simulink model "FCSMPC_double_vector_2025b"  (R2025b)
settings: Solver=FixedStepDiscrete  StartTime=0.0  StopTime=2  FixedStep=SimulinkTs  RelTol=1e-3
PreLoadFcn:
  | % Verzeichnis des Modells zum MATLAB-Pfad hinzufügen
  | modelDir = fileparts(get_param(bdroot, 'FileName'));
  | addpath(modelDir);
  | 
  | % Nur der Dateiname – kein Pfad!
  | set_param(bdroot, 'DataDictionary', 'FOC_params.sldd');
model workspace (MAT data in the model file):
  Np : Simulink.Parameter (value not decoded)
values from neighbouring files (symbols this model uses):
  Filter_Current_FilterTimeConst = 3.3333333333333335E-5    [FOC_params.sldd]
  Filter_Current_SensorTimeConst = 1.5915494309189535E-6    [FOC_params.sldd]
  FOC = evalin("base", "FOC")    [createFOC_SLDD.m]
  FOC_Control_Current_KIid = 10.0    [FOC_params.sldd]
  FOC_Control_Current_KIiq = 10.0    [FOC_params.sldd]
  FOC_Control_Current_KPid = 0.20418507462686566    [FOC_params.sldd]
  FOC_Control_Current_KPiq = 0.58674626865671642    [FOC_params.sldd]
  FOC_Control_Current_Krd = 0.8    [FOC_params.sldd]
  FOC_Control_Current_Krq = 0.8    [FOC_params.sldd]
  FOC_Control_Current_TclCur = 0.1    [FOC_params.sldd]
  FOC_Control_Current_Tnd = 0.1    [FOC_params.sldd]
  FOC_Control_Current_Tnq = 0.1    [FOC_params.sldd]
  FOC_Control_InverterVdc_V = 400.0    [FOC_params.sldd]
  FOC_Control_MotorImax_A = 650.0    [FOC_params.sldd]
  FOC_Control_MTPA_MTPV_nT_id_grid = -450.06704889786266 -439.56177000270145 -427.77784873303676 -416.66404703197372 -406.07553272717422 -395.15516533678584 -384.31176061747851 -374.03652088128132 -363.90551910193739 -353.79478643334204 -344.0221683092833 -334.51243453441936 -324.94614350292119 -315.21793409137081 -305.26543360965195 -295.21828280911944 -285.133916324101 -275.01232812136521 -264.86951532374729 -254.7797625148454 -244    [FOC_params.sldd]
  FOC_Control_MTPA_MTPV_nT_iq_grid = -449.09165648258488 -442.56958748923387 -437.25247759546528 -430.91792082419158 -423.83735797306491 -417.11730433547 -410.54064621830616 -403.71584331167304 -396.93611069310379 -390.15794305727007 -382.97216593027133 -375.44639668848538 -367.93447385667577 -360.57088856352266 -353.41289778449368 -346.34020584402072 -339.28416684923008 -332.22010880540631 -325.11927997033376 -317.92299905654966 -31    [FOC_params.sldd]
  FOC_Control_MTPA_MTPV_T_vec = -245.0 -240.0 -235.0 -230.0 -225.0 -220.0 -215.0 -210.0 -205.0 -200.0 -195.0 -190.0 -185.0 -180.0 -175.0 -170.0 -165.0 -160.0 -155.0 -150.0 -145.0 -140.0 -135.0 -130.0 -125.0 -120.0 -115.0 -110.0 -105.0 -100.0 -95.0 -90.0 -85.0 -80.0 -75.0 -70.0 -65.0 -60.0 -55.0 -50.0 -45.0 -40.0 -35.0 -30.0 -25.0 -20.0 -15.0 -10.0 -5.0 0.0 5.0 10.0 15.0 20.0 25.0 30.0 35.0 40.0 45.0 50.0 55.0 60.0 65.0 70.0 75.0    [FOC_params.sldd]
  FOC_Control_MTPA_MTPV_w_vec = 0.0 10.471975511965978 20.943951023931955 31.415926535897931 41.887902047863911 52.359877559829883 62.831853071795862 73.303828583761828 83.775804095727821 94.247779607693786 104.71975511965977 115.19173063162575 125.66370614359172 136.1356816555577 146.60765716752366 157.07963267948966 167.55160819145564 178.02358370342159 188.49555921538757 198.96753472735358 209.43951023931953 219.9114857512855    [FOC_params.sldd]
  FOC_Control_OpenLoop_Id_Ref_A = 0.0    [FOC_params.sldd]
  FOC_Control_OpenLoop_Iq_Ref_A = 0.0    [FOC_params.sldd]
  FOC_Control_OpenLoop_Ud_OpenLoop_V = 0.0    [FOC_params.sldd]
  FOC_Control_OpenLoop_Uq_OpenLoop_V = 0.0    [FOC_params.sldd]
  FOC_Control_RF_omegamech_rad_s = 3141.5926535897934    [FOC_params.sldd]
  FOC_Control_RF_RateCurrent_A = 500.0    [FOC_params.sldd]
  FOC_Control_RF_RateTrq_Nm = 500.0    [FOC_params.sldd]
  FOC_Control_theta_mechOffsetFix = 0.0    [FOC_params.sldd]
  FOC_Control_theta_mechOffsetTime = 0.0    [FOC_params.sldd]
  FOC_Control_TorqueRef_Nm = 10.0    [FOC_params.sldd]
  FOC_Control_Umax_V = 230.94010767585033    [FOC_params.sldd]
  FOC_Flag_ClosedLoopControl = 1.0    [FOC_params.sldd]
  FOC_Flag_ControlStrategy = 2.0    [FOC_params.sldd]
  FOC_Flag_PWMEnable = 1.0    [FOC_params.sldd]
  FOC_Flag_ResetControl = 0.0    [FOC_params.sldd]
  FOC_Flag_TorqueControl = 1.0    [FOC_params.sldd]
  FOC_LUT_DQLimiter_DQ_LUTScaling = 1.8749999999999995E-5    [FOC_params.sldd]
  FOC_PWM_AZSPWMMethod = 3.0    [FOC_params.sldd]
  FOC_PWM_HybridMode = 1.0    [FOC_params.sldd]
  FOC_PWM_LB1 = 0.5    [FOC_params.sldd]
  FOC_PWM_LB2 = 0.77    [FOC_params.sldd]
  FOC_PWM_PWMManuel = 1.0    [FOC_params.sldd]
  FOC_PWM_RSPWMMethod = 2.0    [FOC_params.sldd]
  FOC_PWM_UB1 = 0.66    [FOC_params.sldd]
  FOC_PWM_UB2 = 0.9    [FOC_params.sldd]
  FOC_SampleTime_TsCur = 0.0001    [FOC_params.sldd]
undefined symbols (not defined in the file or in its folder): dspblkCoreblockFVToolHelper, FCS, Filter, gcbh, Plant, SimulinkTs
libraries: hdlsllib x2, simulink x2, autolibfluxpmsm x1
(part 6 of 8)

== matlab function FCSMPC_double_vector_2025b/FCS_MPC/SDA_Solve/SDA Solve/PSPL_TestFrame/SDA_PL_Framework/QuadraticCalc ==
  data: problem input Bus: SdaProblemBus size=[1 1]; done output boolean size=[1 1]; start input boolean size=[1 1]; level input uint8 size=[1 1]; memory input Bus: SdaMemoryBus size=[1 1]; valid output boolean size=[1 1]; metricNew output double size=[1 1]; head output double size=[1 1]; center output double size=[1 1]; firstCandidate output boolean size=[1 1]; candidate output boolean size=[1 1]; residual output double size=[1 1]
function [done, valid, metricNew, head, center, firstCandidate, candidate, residual] = QuadraticCalc(problem, start, level, memory)
%#codegen
persistent metricReg headReg centerReg firstReg candidateReg residualReg validReg
if isempty(metricReg)
    metricReg=0.0; headReg=0.0; centerReg=0.0;
    firstReg=false; candidateReg=false; residualReg=0.0; validReg=false;
end
done=false;
if start
    idx=max(uint8(1),min(uint8(15),level));
    row=double(idx); headReg=0.0;
    for k=1:15
        if k<row
            headReg=headReg+problem.H(row,k)*double(memory.Uwork(k));
        end
    end
    diagonal=problem.H(row,row);
    validReg=isfinite(diagonal)&&abs(diagonal)>1e-12;
    if validReg
        centerReg=(memory.z(row)-headReg)/diagonal;
        firstReg=centerReg>0.5;
        if memory.candidatePosition(row)==uint8(1)
            candidateReg=firstReg;
        else
            candidateReg=~firstReg;
        end
        residualReg=memory.z(row)-headReg-diagonal*double(candidateReg);
        metricReg=memory.metricStack(row)+residualReg*residualReg;
        validReg=isfinite(centerReg)&&isfinite(metricReg);
    else
        centerReg=0.0; firstReg=false; candidateReg=false;
        residualReg=0.0; metricReg=realmax;
    end
    done=true;
end
valid=validReg; metricNew=metricReg; head=headReg; center=centerReg;
firstCandidate=firstReg; candidate=candidateReg; residual=residualReg;
end

== matlab function FCSMPC_double_vector_2025b/FCS_MPC/SDA_Solve/SDA Solve/PSPL_TestFrame/SDA_PL_Framework/ResultCommit ==
  data: problem input Bus: SdaProblemBus size=[1 1]; result output Bus: SdaResultBus size=[1 1]; commit input boolean size=[1 1]; best input Bus: SdaBestBus size=[1 1]; nodes input uint32 size=[1 1]; leafNodes input uint32 size=[1 1]; nodeLimitReached input boolean size=[1 1]; Jround input double size=[1 1]; Jshift input double size=[1 1]
function result = ResultCommit(problem,commit,best,nodes,leafNodes,nodeLimitReached,Jround,Jshift)
%#codegen
persistent state
if isempty(state)
 state.valid=false; state.Jopt=realmax; state.nodes=uint32(0);
 state.optimal=false; state.Uopt=zeros(15,1); state.Uapply=zeros(6,1);
 state.leafNodes=uint32(0); state.bestCMVCost=0.0; state.cmvMetricRatio=0.0;
 state.switchCountApplied=uint32(0); state.debugLower=zeros(3,1);
 state.debugUpper=zeros(3,1); state.iabcPredictedNext=zeros(3,1);
 state.Jround=0.0; state.Jshift=0.0; state.predictionValidNext=false; state.solutionToggle=false;
end
if commit
 state.valid=best.bestValid; state.Jopt=best.bestMetric;
 state.nodes=nodes; state.leafNodes=leafNodes;
 state.optimal=best.bestValid&&~nodeLimitReached;
 state.Uopt=double(best.bestU); state.Uapply=state.Uopt(1:6);
 state.bestCMVCost=best.bestCMVCost;
 if state.Jopt>eps, state.cmvMetricRatio=state.bestCMVCost/state.Jopt; else, state.cmvMetricRatio=0.0; end
 sPrev=problem.UoptPrev(4:6); sFirst=state.Uopt(1:3); sSecond=state.Uopt(4:6);
 [deltaFirst,deltaDead]=deadtime_step(sPrev,sFirst,problem.iabcCompensated,problem);
 iabcAfter=problem.iabcCompensated+deltaFirst;
 [deltaSecond,~]=deadtime_step(sFirst,sSecond,iabcAfter,problem);
 state.iabcPredictedNext=iabcAfter+deltaSecond;
 state.switchCountApplied=uint32(sum(abs(sFirst-sPrev))+sum(abs(sSecond-sFirst)));
 [~,state.debugLower,state.debugUpper]=cmv_bounds(problem.iabcCompensated,deltaDead,problem.currentEpsMargin);
 state.Jround=Jround; state.Jshift=Jshift; state.predictionValidNext=best.bestValid;
 state.solutionToggle=~state.solutionToggle;
end
result=state;
end

function [deltaStep,deltaDead]=deadtime_step(sPrevious,sCurrent,iabc,problem)
sDead=sCurrent; signEps=0.1*problem.currentEpsMargin;
for phase=1:3
 if sPrevious(phase)~=sCurrent(phase)
  if iabc(phase)>=signEps, sDead(phase)=0.0;
  elseif iabc(phase)<=-signEps, sDead(phase)=1.0;
  elseif signEps>0.0, sDead(phase)=0.5*(1.0-iabc(phase)/signEps);
  else, sDead(phase)=0.5; end
 end
end
sEffective=problem.deadtimeRatio*sDead+(1.0-problem.deadtimeRatio)*sCurrent;
deltaDead=problem.deadtimeRatio*(problem.deltaIabcBase+problem.deltaIabcSwitch*sDead);
deltaStep=problem.deltaIabcBase+problem.deltaIabcSwitch*sEffective;
end

function [iabcEnd,lower,upper]=cmv_bounds(iabc,deltaDead,margin)
iabcEnd=iabc+deltaDead; lower=min(iabc,iabcEnd)-margin; upper=max(iabc,iabcEnd)+margin;
end

== matlab function FCSMPC_double_vector_2025b/FCS_MPC/SDA_Solve/SDA Solve/PSPL_TestFrame/SDA_PL_Framework/SdaInitializer ==
  data: problem input Bus: SdaProblemBus size=[1 1]; done output boolean size=[1 1]; start input boolean size=[1 1]; valid output boolean size=[1 1]; z output double size=[15 1]; initialU output double size=[15 1]; initialMetric output double size=[1 1]; initialCMVCost output double size=[1 1]; Jround output double size=[1 1]; Jshift output double size=[1 1]
function [done, valid, z, initialU, initialMetric, initialCMVCost, Jround, Jshift] = SdaInitializer(problem, start)
%#codegen
persistent zReg uReg metricReg cmvReg jRoundReg jShiftReg validReg
if isempty(zReg)
    zReg=zeros(15,1); uReg=zeros(15,1); metricReg=realmax;
    cmvReg=0.0; jRoundReg=0.0; jShiftReg=0.0; validReg=false;
end
done=false;
if start
    zReg=problem.H*problem.U_unc;
    uRound=zeros(15,1); uShift=zeros(15,1);
    for k=1:15
        uRound(k)=min(max(round(problem.U_unc(k)),0.0),1.0);
    end
    for k=1:12
        uShift(k)=problem.UoptPrev(k+3);
    end
    for k=13:15
        uShift(k)=problem.UoptPrev(k);
    end
    jRoundReg=quadratic_cost(problem.H,uRound,problem.U_unc);
    jShiftReg=quadratic_cost(problem.H,uShift,problem.U_unc);
    if jShiftReg < jRoundReg
        uReg=uShift;
    else
        uReg=uRound;
    end
    sPrevious=problem.UoptPrev(4:6);
    cmvReg=sequence_cmv_cost(uReg,sPrevious,problem);
    metricReg=quadratic_cost(problem.H,uReg,problem.U_unc)+cmvReg;
    validReg=isfinite(metricReg);
    done=true;
end
valid=validReg; z=zReg; initialU=uReg; initialMetric=metricReg;
initialCMVCost=cmvReg; Jround=jRoundReg; Jshift=jShiftReg;
end

function value=quadratic_cost(H,U,Uunc)
residual=H*(U-Uunc);
value=norm(residual,2)^2;
end

function total=sequence_cmv_cost(U,sPrevious,problem)
total=0.0; iabc=problem.iabcCompensated;
for step=1:5
    first=(step-1)*3+1; sCurrent=U(first:first+2);
    [deltaStep,deltaDead]=deadtime_step(sPrevious,sCurrent,iabc,problem);
    total=total+cmv_penalty(sPrevious,sCurrent,iabc,deltaDead,problem);
    iabc=iabc+deltaStep; sPrevious=sCurrent;
end
end

function [deltaStep,deltaDead]=deadtime_step(sPrevious,sCurrent,iabc,problem)
sDead=sCurrent; signEps=0.1*problem.currentEpsMargin;
for phase=1:3
    if sPrevious(phase)~=sCurrent(phase)
        if iabc(phase)>=signEps
            sDead(phase)=0.0;
        elseif iabc(phase)<=-signEps
            sDead(phase)=1.0;
        elseif signEps>0.0
            sDead(phase)=0.5*(1.0-iabc(phase)/signEps);
        else
            sDead(phase)=0.5;
        end
    end
end
sEffective=problem.deadtimeRatio*sDead+(1.0-problem.deadtimeRatio)*sCurrent;
deltaDead=problem.deadtimeRatio*(problem.deltaIabcBase+problem.deltaIabcSwitch*sDead);
deltaStep=problem.deltaIabcBase+problem.deltaIabcSwitch*sEffective;
end

function penalty=cmv_penalty(sPrevious,sCurrent,iabc,deltaDead,problem)
penalty=0.0; iabcEnd=iabc+deltaDead;
lower=min(iabc,iabcEnd)-problem.currentEpsMargin;
upper=max(iabc,iabcEnd)+problem.currentEpsMargin;
uncertain=(lower<=0.0)&(upper>=0.0);
if all(sCurrent==0.0)||all(sCurrent==1.0)
    penalty=penalty+problem.lambdaZero;
end
changed=(sPrevious~=sCurrent);
if sum(changed)~=2
    return;
end
canZero=false(3,1); canOne=false(3,1);
for phase=1:3
    if ~changed(phase)
        canZero(phase)=sPrevious(phase)==0.0;
        canOne(phase)=sPrevious(phase)==1.0;
    elseif uncertain(phase)
        canZero(phase)=true; canOne(phase)=true;
    elseif iabcEnd(phase)>0.0
        canZero(phase)=true;
    else
        canOne(phase)=true;
    end
end
if all(canZero)||all(canOne)
    penalty=penalty+problem.lambdaDeadtime;
end
end

== matlab function FCSMPC_double_vector_2025b/FCS_MPC/SDA_Solve/SDA Solve/PSPL_TestFrame/SDA_PL_Framework/SearchCounter ==
  data: clear input boolean size=[1 1]; nodes output uint32 size=[1 1]; writeEnable input boolean size=[1 1]; fsmState input uint8 size=[1 1]; level input uint8 size=[1 1]; problem input Bus: SdaProblemBus size=[1 1]; leafNodes output uint32 size=[1 1]; nodeLimitReached output boolean size=[1 1]; currentPrune input boolean size=[1 1]
function [nodes,leafNodes,nodeLimitReached] = SearchCounter(clear,writeEnable,fsmState,level,problem,currentPrune)
%#codegen
persistent nodeReg leafReg limitReg leafStatePrev
if isempty(nodeReg), nodeReg=uint32(0); leafReg=uint32(0); limitReg=false; leafStatePrev=false; end
if clear, nodeReg=uint32(0); leafReg=uint32(0); limitReg=false; leafStatePrev=false; end
if writeEnable&&fsmState==uint8(7)
 nodeReg=nodeReg+uint32(1);
 if problem.NmaxNode>uint32(0)&&nodeReg>problem.NmaxNode, limitReg=true; end
end
leafStateNow=fsmState==uint8(16);
if leafStateNow&&~leafStatePrev&&level==uint8(15)&&~currentPrune
 leafReg=leafReg+uint32(1);
end
leafStatePrev=leafStateNow;
nodes=nodeReg; leafNodes=leafReg; nodeLimitReached=limitReg;
end

== stateflow chart FCSMPC_double_vector_2025b/FCS_MPC/SDA_Solve/SDA Solve/PSPL_TestFrame/SDA_PL_Framework/SearchFSM ==
  settings: updateMethod=DISCRETE
  state IDLE
    entry: level=uint8(1); candidate=false; cycleCount=uint32(0); busy=false; resultValid=false; fault=false;
  state DONE
    entry: loadProblem=false; initStart=false; quadStart=false; vectorStart=false; memClear=false; memWrite=false; bestWrite=false; commitResult=false; busy=false; resultValid=true; fault=false;
  state FAULT
    entry: busy=false; fault=true;
  state LOAD
    entry: busy=true; loadProblem=true; memClear=true; level=uint8(1); cycleCount=uint32(0);
  state CENTER_WAIT
    during: loadProblem=false; initStart=false; quadStart=false; vectorStart=false; memClear=false; memWrite=false; bestWrite=false; commitResult=false; resultValid=false; fault=false; fsmState=uint8(6); cycleCount=cycleCount+uint32(1);
  state WRITE_RESULT
    entry: commitResult=true;
  state INIT_START
    entry: initStart=true;
  state INIT_WAIT
    during: loadProblem=false; initStart=false; quadStart=false; vectorStart=false; memClear=false; memWrite=false; bestWrite=false; commitResult=false; resultValid=false; fault=false; fsmState=uint8(3); cycleCount=cycleCount+uint32(1);
  state CENTER_START
    entry: quadStart=true;
  state SELECT_CANDIDATE
    entry: fsmState=uint8(7); candidate=quadCandidate; memWrite=true;
  state BACKTRACK
    entry: fsmState=uint8(17); if level>uint8(0); level=level-uint8(1); end; memWrite=true;
  state CHECK_LEVEL
    entry: loadProblem=false; initStart=false; quadStart=false; vectorStart=false; memClear=false; memWrite=false; bestWrite=false; commitResult=false; resultValid=false; fault=false; fsmState=uint8(4); cycleCount=cycleCount+uint32(1);
  state VECTOR_WAIT
    during: loadProblem=false; initStart=false; quadStart=false; vectorStart=false; memClear=false; memWrite=false; bestWrite=false; commitResult=false; resultValid=false; fault=false; fsmState=uint8(12); cycleCount=cycleCount+uint32(1);
  state NEXT_CANDIDATE
    entry: loadProblem=false; initStart=false; quadStart=false; vectorStart=false; memClear=false; memWrite=false; bestWrite=false; commitResult=false; resultValid=false; fault=false; fsmState=uint8(16); cycleCount=cycleCount+uint32(1);
  state DESCEND
    entry: fsmState=uint8(15); level=level+uint8(1); memWrite=true;
  state VECTOR_START
    entry: vectorStart=true;
  state VECTOR_CHECK
    entry: loadProblem=false; initStart=false; quadStart=false; vectorStart=false; memClear=false; memWrite=false; bestWrite=false; commitResult=false; resultValid=false; fault=false; fsmState=uint8(10); cycleCount=cycleCount+uint32(1);
  state UPDATE_BEST
    entry: bestWrite=true;
  state COMPARE
    entry: loadProblem=false; initStart=false; quadStart=false; vectorStart=false; memClear=false; memWrite=false; bestWrite=false; commitResult=false; resultValid=false; fault=false; fsmState=uint8(13); cycleCount=cycleCount+uint32(1);
  (default) -> IDLE
  DONE -> IDLE
  FAULT -> IDLE : [~start]
  IDLE -> LOAD : [start]
  CENTER_WAIT -> FAULT [order 2] : [quadDone && ~quadValid]
  WRITE_RESULT -> DONE
  INIT_WAIT -> FAULT [order 2] : [initDone && ~initValid]
  VECTOR_WAIT -> FAULT [order 2] : [vectorDone && ~vectorValid]
  LOAD -> INIT_START
  CENTER_WAIT -> SELECT_CANDIDATE [order 1] : [quadDone && quadValid]
  CENTER_START -> CENTER_WAIT
  INIT_START -> INIT_WAIT
  BACKTRACK -> WRITE_RESULT [order 2] : [level==uint8(0)]
  CHECK_LEVEL -> WRITE_RESULT [order 3] : [nodeLimitReached]
  INIT_WAIT -> CHECK_LEVEL [order 1] : [initDone && initValid]
  SELECT_CANDIDATE -> VECTOR_CHECK
  CHECK_LEVEL -> CENTER_START [order 1] : [~nodeLimitReached && ~candidateExhausted]
  CHECK_LEVEL -> BACKTRACK [order 2] : [~nodeLimitReached && candidateExhausted]
  BACKTRACK -> CHECK_LEVEL [order 1] : [level>uint8(0)]
  NEXT_CANDIDATE -> CHECK_LEVEL
  DESCEND -> CHECK_LEVEL
  VECTOR_WAIT -> COMPARE [order 1] : [vectorDone && vectorValid]
  VECTOR_START -> VECTOR_WAIT
  COMPARE -> NEXT_CANDIDATE [order 3] : [currentPrune || (level==uint8(15) && ~currentBetter)]
  UPDATE_BEST -> NEXT_CANDIDATE
  COMPARE -> DESCEND [order 2] : [level<uint8(15) && ~currentPrune]
  VECTOR_CHECK -> VECTOR_START [order 1] : [mod(level,uint8(3))==0]
  VECTOR_CHECK -> COMPARE [order 2] : [mod(level,uint8(3))~=0]
  COMPARE -> UPDATE_BEST [order 1] : [level==uint8(15) && currentBetter]
  data: start input boolean size=[1 1]; initDone input boolean size=[1 1]; initValid input boolean size=[1 1]; quadDone input boolean size=[1 1]; quadValid input boolean size=[1 1]; vectorDone input boolean size=[1 1]; vectorValid input boolean size=[1 1]; loadProblem output boolean size=[1 1]; initStart output boolean size=[1 1]; quadStart output boolean size=[1 1]; vectorStart output boolean size=[1 1]; memClear output boolean size=[1 1]; memWrite output boolean size=[1 1]; bestWrite output boolean size=[1 1]; commitResult output boolean size=[1 1]; busy output boolean size=[1 1]; resultValid output boolean size=[1 1]; fault output boolean size=[1 1]; level output uint8 size=[1 1]; candidate output boolean size=[1 1]; fsmState output uint8 size=[1 1]; cycleCount output uint32 size=[1 1]; quadCandidate input boolean size=[1 1]; candidateExhausted input boolean size=[1 1]; currentBetter input boolean size=[1 1]; currentPrune input boolean size=[1 1]; nodeLimitReached input boolean size=[1 1]

== matlab function FCSMPC_double_vector_2025b/FCS_MPC/SDA_Solve/SDA Solve/PSPL_TestFrame/SDA_PL_Framework/VectorCostCalc ==
  data: problem input Bus: SdaProblemBus size=[1 1]; done output boolean size=[1 1]; start input boolean size=[1 1]; level input uint8 size=[1 1]; memory input Bus: SdaMemoryBus size=[1 1]; valid output boolean size=[1 1]; totalMetricNew output double size=[1 1]; cmvMetricNew output double size=[1 1]; cmvIncrement output double size=[1 1]; iabcNext output double size=[3 1]; deltaStep output double size=[3 1]; deltaDead output double size=[3 1]; lowerBound output double size=[3 1]; upperBound output double size=[3 1]; deadtimeMiss output boolean size=[1 1]
function [done,valid,totalMetricNew,cmvMetricNew,cmvIncrement,iabcNext,deltaStep,deltaDead,lowerBound,upperBound,deadtimeMiss] = VectorCostCalc(problem,start,level,memory)
%#codegen
persistent totalReg cmvTotalReg incrementReg iabcReg stepReg deadReg lowerReg upperReg missReg validReg startPrev doneReg
if isempty(totalReg)
    totalReg=0.0; cmvTotalReg=0.0; incrementReg=0.0;
    iabcReg=zeros(3,1); stepReg=zeros(3,1); deadReg=zeros(3,1);
    lowerReg=zeros(3,1); upperReg=zeros(3,1);
    missReg=false; validReg=false; startPrev=false; doneReg=false;
end
done=doneReg;
if start&&~startPrev
    idx=max(uint8(3),min(uint8(15),level));
    predictionStep=idivide(idx,uint8(3));
    blockEnd=double(idx); blockStart=blockEnd-2;
    sCurrent=zeros(3,1); sPrevious=zeros(3,1);
    for phase=1:3
        sCurrent(phase)=double(memory.Uwork(blockStart+phase-1));
    end
    if predictionStep==uint8(1)
        sPrevious=problem.UoptPrev(4:6);
    else
        previousStart=blockStart-3;
        for phase=1:3
            sPrevious(phase)=double(memory.Uwork(previousStart+phase-1));
        end
    end
    iabcBefore=memory.iabcPrediction(:,double(predictionStep));
    [stepReg,deadReg]=deadtime_step(sPrevious,sCurrent,iabcBefore,problem);
    [incrementReg,lowerReg,upperReg,missReg]=cmv_penalty(sPrevious,sCurrent,iabcBefore,deadReg,problem);
    totalReg=memory.metricStack(double(idx)+1)+incrementReg;
    cmvTotalReg=memory.cmvMetricStack(double(idx))+incrementReg;
    iabcReg=iabcBefore+stepReg;
    validReg=all(isfinite(iabcReg))&&isfinite(totalReg)&&isfinite(cmvTotalReg);
    doneReg=true;
end
if ~start&&~startPrev, doneReg=false; end
startPrev=start;
valid=validReg; totalMetricNew=totalReg; cmvMetricNew=cmvTotalReg;
cmvIncrement=incrementReg; iabcNext=iabcReg; deltaStep=stepReg;
deltaDead=deadReg; lowerBound=lowerReg; upperBound=upperReg;
deadtimeMiss=missReg;
end

function [deltaStep,deltaDead]=deadtime_step(sPrevious,sCurrent,iabc,problem)
sDead=sCurrent; signEps=0.1*problem.currentEpsMargin;
for phase=1:3
    if sPrevious(phase)~=sCurrent(phase)
        if iabc(phase)>=signEps
            sDead(phase)=0.0;
        elseif iabc(phase)<=-signEps
            sDead(phase)=1.0;
        elseif signEps>0.0
            sDead(phase)=0.5*(1.0-iabc(phase)/signEps);
        else
            sDead(phase)=0.5;
        end
    end
end
sEffective=problem.deadtimeRatio*sDead+(1.0-problem.deadtimeRatio)*sCurrent;
deltaDead=problem.deadtimeRatio*(problem.deltaIabcBase+problem.deltaIabcSwitch*sDead);
deltaStep=problem.deltaIabcBase+problem.deltaIabcSwitch*sEffective;
end

function [penalty,lower,upper,deadtimeMiss]=cmv_penalty(sPrevious,sCurrent,iabc,deltaDead,problem)
penalty=0.0; deadtimeMiss=false; iabcEnd=iabc+deltaDead;
lower=min(iabc,iabcEnd)-problem.currentEpsMargin;
upper=max(iabc,iabcEnd)+problem.currentEpsMargin;
uncertain=(lower<=0.0)&(upper>=0.0);
if all(sCurrent==0.0)||all(sCurrent==1.0)
    penalty=penalty+problem.lambdaZero;
end
changed=(sPrevious~=sCurrent);
if sum(changed)==2
    canZero=false(3,1); canOne=false(3,1);
    for phase=1:3
        if ~changed(phase)
            canZero(phase)=sPrevious(phase)==0.0;
            canOne(phase)=sPrevious(phase)==1.0;
        elseif uncertain(phase)
            canZero(phase)=true; canOne(phase)=true;
        elseif iabcEnd(phase)>0.0
            canZero(phase)=true;
        else
            canOne(phase)=true;
        end
    end
    deadtimeMiss=all(canZero)||all(canOne);
    if deadtimeMiss
        penalty=penalty+problem.lambdaDeadtime;
    end
end
end

== matlab function FCSMPC_double_vector_2025b/FCS_MPC/BuildModel/BuildModel/QP_Precompute_10k_Simplified_hybrid ==
  data: Ld input double size=[1 1]; H_exp output double size=[15 15]; H_emb output; Lq input double size=[1 1]; Rs input double size=[1 1]; Psi input double size=[1 1]; wel input double size=[1 1]; Ts input double size=[1 1]; Vdc input double size=[1 1]; lambda_fsw input double size=[1 1]; lambdaZeroEmbedded input; Sin_Cos_Theta input double size=[2 1]; filterTimeConstant input double size=[1 1]; sensorTimeConstant input double size=[1 1]; Gamma output double size=[10 2]; Phi output double size=[10 1]; Lambdafsw_SE output double size=[15 3]; Upsil output double size=[10 15]; Bd output double size=[2 2]; Bs_TI output double size=[2 3]; deltaIdqBaseOffset output double size=[2 1]; deltaIdqState output double size=[2 2]; magnitudeGain output double size=[1 1]; phaseCompensation output double size=[2 2]; rippleAttenuation output double size=[1 1]; rippleDelay output double size=[1 1]
function [H_exp,H_emb,Gamma,Phi,Lambdafsw_SE,Upsil, ...
    Bd,Bs_TI,deltaIdqBaseOffset,deltaIdqState, ...
    magnitudeGain,phaseCompensation,rippleAttenuation,rippleDelay] = ...
    QP_Precompute_10k_Simplified_Hybrid( ...
    Ld,Lq,Rs,Psi,wel,Ts,Vdc,lambda_fsw,lambdaZeroEmbedded, ...
    Sin_Cos_Theta,filterTimeConstant,sensorTimeConstant)
%#codegen
%QP_PRECOMPUTE_10K_SIMPLIFIED_HYBRID Standalone hybrid precomputation.
% H_exp is used by explicit pruning. H_emb includes the exact quadratic
% zero-vector term and is used only for embedded Babai initialization.

Np = 5; nu = 3; ny = 2;
Ts = max(realmin('double'),double(Ts));
filterTimeConstant = max(0.0,double(filterTimeConstant));
sensorTimeConstant = max(0.0,double(sensorTimeConstant));
lambdaZeroEmbedded = max(0.0,double(lambdaZeroEmbedded));

Ac = [-Rs/Ld, wel*Lq/Ld; -wel*Ld/Lq, -Rs/Lq];
Bc = [1/Ld, 0; 0, 1/Lq];
fc = [0; -wel*Psi/Lq];
M = [Ac, Bc, fc; zeros(3,5)];
Md = expm(M*Ts);
Ad = Md(1:2,1:2); Bd = Md(1:2,3:4); fd = Md(1:2,5);

Apow = zeros(ny*(Np+1),ny); Apow(1:ny,:) = eye(ny);
for m = 1:Np
    Apow(m*ny+(1:ny),:) = Apow((m-1)*ny+(1:ny),:)*Ad;
end
Gamma = zeros(ny*Np,ny); Phi = zeros(ny*Np,1);
for i = 1:Np
    rows = (i-1)*ny+(1:ny);
    Gamma(rows,:) = Apow(i*ny+(1:ny),:);
    acc = zeros(ny,1);
    for m = 0:i-1
        acc = acc+Apow(m*ny+(1:ny),:)*fd;
    end
    Phi(rows) = acc;
end

S = eye(nu*Np);
for i = 2:Np
    S((i-1)*nu+(1:nu),(i-2)*nu+(1:nu)) = -eye(nu);
end
E = [eye(nu); zeros(nu*(Np-1),nu)];
lambdaEffective = max(lambda_fsw,1.0e-6);
Lambdafsw_SE = lambdaEffective*(S.'*E);
Lambdafsw_Ssquare = lambdaEffective*(S.'*S);

sinTheta = Sin_Cos_Theta(1); cosTheta = Sin_Cos_Theta(2);
deltaTheta = wel*50.0e-6;
sinDelta = sin(deltaTheta); cosDelta = cos(deltaTheta);
sinMid = sinTheta*cosDelta+cosTheta*sinDelta;
cosMid = cosTheta*cosDelta-sinTheta*sinDelta;
RpMid = [cosMid, sinMid; -sinMid, cosMid];
Msw = eye(3)-ones(3)/3;
Tc = (2/3)*[1, -1/2, -1/2; 0, sqrt(3)/2, -sqrt(3)/2];
Bs_TI = Tc*Vdc*Msw;
deltaIdqSwitchMid = Bd*RpMid*Bs_TI;
Jrot = [0 -1; 1 0];
deltaIdqState = Ad-eye(2)+Jrot*(wel*Ts);
deltaIdqBaseOffset = fd;

Upsil = zeros(ny*Np,nu*Np);
for i = 1:Np
    rows = (i-1)*ny+(1:ny);
    for j = 1:i
        cols = (j-1)*nu+(1:nu);
        Upsil(rows,cols) = ...
            Apow((i-j)*ny+(1:ny),:)*deltaIdqSwitchMid;
    end
end

W_exp = Upsil.'*Upsil+Lambdafsw_Ssquare;
WzeroEmbedded = 0.5*lambdaZeroEmbedded*kron(eye(Np),ones(nu));
H_exp = reversed_cholesky(W_exp);
H_emb = reversed_cholesky(W_exp+WzeroEmbedded);

omegaFilter = wel*filterTimeConstant;
omegaSensor = wel*sensorTimeConstant;
magnitudeGain = sqrt(1.0+omegaFilter*omegaFilter)* ...
    sqrt(1.0+omegaSensor*omegaSensor);
w = abs(wel);
if w > 1.0e-6
    basePhaseDelay = (atan(w*filterTimeConstant)+ ...
        atan(w*sensorTimeConstant))/w;
else
    basePhaseDelay = filterTimeConstant+sensorTimeConstant;
end
phase = wel*basePhaseDelay;
phaseCompensation = [cos(phase), -sin(phase); sin(phase), cos(phase)];
omegaRipple = 2.0*pi*17.0e3;
xFilter = omegaRipple*filterTimeConstant;
xSensor = omegaRipple*sensorTimeConstant;
rippleAttenuation = 1.0/(sqrt(1.0+xFilter*xFilter)* ...
    sqrt(1.0+xSensor*xSensor));
rippleDelay = (atan(xFilter)+atan(xSensor))/omegaRipple;
rippleDelay = min(max(0.0,rippleDelay),2.0*Ts);
end

function H = reversed_cholesky(W)
n = size(W,1);
W = 0.5*(W+W.');
W = W+1.0e-12*max(1.0,norm(W,'fro'))*eye(n);
Jx = fliplr(eye(n));
[Rt,p] = chol(Jx*W*Jx);
if p ~= 0
    error('Hessian is not positive definite. Increase lambda_sw.');
end
H = Jx*Rt*Jx;
end

== matlab function FCSMPC_double_vector_2025b/FCS_MPC/SDA_Solve/SDA Solve/direct_feedthrough ==
  data: Ad input size=[2 2]; iabcReconstruction output size=[3 1]; Bd input size=[2 2]; fd input size=[2 1]; Bs_TI input size=[2 3]; idiqFiltered input size=[2 1]; Sin_Cos_Theta input size=[2 1]; wel input size=1; Ts input size=1; U_applied input size=[6 1]; controllerDelay input size=1; iabcPredictedPrevious input size=[3 1]; Iabc_Motor input size=[3 1]; predictionValid input; filterTimeConstant input; sensorTimeConstant input; filterDelayGain input; idiqCompensated output size=[2 1]; deltaIabcBase output size=[3 1]; deltaIabcSwitch output size=[3 3]; Bs output size=[2 3]; predictionError output size=[3 1]; reconstructionError output size=[3 1]; predictionError_dq output; reconstructionError_dq output; iabcAverageEstimated output size=[3 1]; iabcRippleEstimated output size=[3 1]; rippleResidual output; iabcSwitchCorrectionRaw output
function [iabcReconstruction,idiqCompensated, ...
    deltaIabcBase,deltaIabcSwitch,Bs, ...
    predictionError,reconstructionError, ...
    predictionError_dq,reconstructionError_dq, ...
    iabcAverageEstimated,iabcRippleEstimated,rippleResidual, ...
    iabcSwitchCorrectionRaw] = ...
    Current_Reconstruction_Direct_Feedthrough( ...
    Ad,Bd,fd,Bs_TI,idiqFiltered, ...
    Sin_Cos_Theta,wel,Ts,U_applied,controllerDelay, ...
    iabcPredictedPrevious,Iabc_Motor,predictionValid, ...
    filterTimeConstant,sensorTimeConstant,filterDelayGain) %#ok<INUSD>
%CURRENT_RECONSTRUCTION_DIRECT_FEEDTHROUGH Ideal-current baseline for SDA.
%#codegen
%
% This variant bypasses the sensor/filter reconstruction and feeds the
% simulated motor phase current directly to SDA:
%   iabcReconstruction = Iabc_Motor.
% It isolates SDA prediction/search performance from reconstruction error.
%
% IMPORTANT: Iabc_Motor is available in simulation but is not an
% independently measurable signal in the real controller. This variant is
% therefore intended for benchmarking and diagnosis, not deployment.
%
% Ts is the duration of one SDA vector step and equals 0.5*MPC_Ts in the
% Simulink model. Ad, Bd and fd must be discretized with this same Ts.
%
% Input dimensions:
%   Ad, Bd                    2x2
%   fd                        2x1
%   Bs_TI                     2x3
%   idiqFiltered              2x1 (unused; retained for variant interface)
%   Sin_Cos_Theta             2x1 = [sin(theta); cos(theta)]
%   U_applied                 6x1 (unused; retained for variant interface)
%   iabcPredictedPrevious     3x1
%   Iabc_Motor                3x1
%   all remaining inputs      scalar
%
% Output dimensions:
%   iabcReconstruction        3x1
%   idiqCompensated           2x1
%   deltaIabcBase             3x1
%   deltaIabcSwitch           3x3
%   Bs                        2x3
%   predictionError           3x1
%   reconstructionError       3x1
%   predictionError_dq        2x1
%   reconstructionError_dq    2x1
%   iabcAverageEstimated      3x1
%   iabcRippleEstimated       3x1
%   rippleResidual            3x1
%   iabcSwitchCorrectionRaw   3x1

Ad = double(Ad);
Bd = double(Bd);
fd = double(fd);
Bs_TI = double(Bs_TI);
Sin_Cos_Theta = double(Sin_Cos_Theta);
wel = double(wel);
Ts = max(realmin('double'),double(Ts));
iabcPredictedPrevious = double(iabcPredictedPrevious);
Iabc_Motor = double(Iabc_Motor);

% idiqFiltered, U_applied, controllerDelay, filterTimeConstant,
% sensorTimeConstant and filterDelayGain are intentionally unused. They are
% retained at their original positions so this diagnostic baseline can be
% selected without changing any MATLAB Function block wiring.

sinTheta = Sin_Cos_Theta(1);
cosTheta = Sin_Cos_Theta(2);
Tclarke = [2/3, -1/3, -1/3; ...
           0, 1/sqrt(3), -1/sqrt(3)];
Rpark = [cosTheta, sinTheta; -sinTheta, cosTheta];
TinvClarke = [1.0, 0.0; ...
             -0.5, sqrt(3)/2; ...
             -0.5, -sqrt(3)/2];
Tdq2abc = TinvClarke*Rpark.';

% Ideal current path used by SDA.
iabcReconstruction = Iabc_Motor;
idiqCompensated = Rpark*(Tclarke*iabcReconstruction);

% One-vector-step current increments used by Assembly_QP and SDA_Solve.
Jrot = [0 -1; 1 0];
Bs = Bd*Rpark*Bs_TI;
deltaIdqBase = (Ad-eye(2))*idiqCompensated+fd;
deltaIabcBase = Tdq2abc*( ...
    deltaIdqBase+Jrot*idiqCompensated*(wel*Ts));
deltaIabcSwitch = Tdq2abc*Bs;

% Prediction error remains observable for assessment of the SDA/model
% prediction made in the preceding vector step.
if logical(predictionValid)
    predictionError = iabcReconstruction-iabcPredictedPrevious;
else
    predictionError = zeros(3,1);
end
predictionError_dq = Rpark*(Tclarke*predictionError);

% Direct feedthrough is, by definition, identical to the simulation truth.
reconstructionError = Iabc_Motor-iabcReconstruction;
reconstructionError_dq = Rpark*(Tclarke*reconstructionError);

% Diagnostics that belong to filter/ripple reconstruction are disabled.
iabcAverageEstimated = iabcReconstruction;
iabcRippleEstimated = zeros(3,1);
rippleResidual = zeros(3,1);
iabcSwitchCorrectionRaw = zeros(3,1);
end

== matlab function FCSMPC_double_vector_2025b/FCS_MPC/SDA_Solve/SDA Solve/No_Compensation ==
  data: Ad input size=[2 2]; iabcReconstruction output size=[3 1]; Bd input size=[2 2]; fd input size=[2 1]; Bs_TI input size=[2 3]; idiqFiltered input size=[2 1]; Sin_Cos_Theta input size=[2 1]; wel input size=1; Ts input size=1; U_applied input size=[6 1]; controllerDelay input size=1; iabcPredictedPrevious input size=[3 1]; Iabc_Motor input size=[3 1]; predictionValid input; filterTimeConstant input; sensorTimeConstant input; filterDelayGain input; idiqCompensated output size=[2 1]; deltaIabcBase output size=[3 1]; deltaIabcSwitch output size=[3 3]; Bs output size=[2 3]; predictionError output size=[3 1]; reconstructionError output size=[3 1]; predictionError_dq output; reconstructionError_dq output; iabcAverageEstimated output size=[3 1]; iabcRippleEstimated output size=[3 1]; rippleResidual output; iabcSwitchCorrectionRaw output
function [iabcReconstruction,idiqCompensated, ...
    deltaIabcBase,deltaIabcSwitch,Bs, ...
    predictionError,reconstructionError, ...
    predictionError_dq,reconstructionError_dq, ...
    iabcAverageEstimated,iabcRippleEstimated,rippleResidual, ...
    iabcSwitchCorrectionRaw] = ...
    Current_Reconstruction_No_Compensation( ...
    Ad,Bd,fd,Bs_TI,idiqFiltered, ...
    Sin_Cos_Theta,wel,Ts,U_applied,controllerDelay, ...
    iabcPredictedPrevious,Iabc_Motor,predictionValid, ...
    filterTimeConstant,sensorTimeConstant,filterDelayGain) %#ok<INUSD>
%CURRENT_RECONSTRUCTION_NO_COMPENSATION Uncompensated diagnostic baseline.
%#codegen
% The 16-input/13-output interface exactly matches
% Current_Reconstruction_Switch_Frequency_kHz and its simplified variant.
% idiqFiltered is passed through directly; abc current is obtained only by
% inverse Park and inverse Clarke transforms. No filter, ripple, or
% controller-delay compensation is applied.
% U_applied, controllerDelay,
% filterTimeConstant, sensorTimeConstant, and filterDelayGain are retained
% for interface compatibility and are intentionally unused.
% Prediction error uses the same validity gate and dq transform as hybrid.
% Ripple/correction diagnostics are disabled (zero).
% iabcAverageEstimated is the uncorrected transformed measurement.

Ad = double(Ad);
Bd = double(Bd);
fd = double(fd);
Bs_TI = double(Bs_TI);
idiqFiltered = double(idiqFiltered);
Sin_Cos_Theta = double(Sin_Cos_Theta);
wel = double(wel);
Ts = max(realmin('double'),double(Ts));
iabcPredictedPrevious = double(iabcPredictedPrevious);
Iabc_Motor = double(Iabc_Motor);
predictionValid = logical(predictionValid);
% Ts is the SDA vector-step duration supplied as 0.5*MPC_Ts. The discrete
% matrices and the increments exported to SDA use this same time base.

sinTheta = Sin_Cos_Theta(1);
cosTheta = Sin_Cos_Theta(2);
Rpark = [cosTheta, sinTheta; -sinTheta, cosTheta];
TinvClarke = [1.0, 0.0; ...
             -0.5, sqrt(3)/2; ...
             -0.5, -sqrt(3)/2];
Tdq2abc = TinvClarke*Rpark.';

idiqCompensated = idiqFiltered;
idiqState = idiqFiltered;
iabcReconstruction = Tdq2abc*idiqState;

% Preserve the original one-vector-step current-increment model, evaluated directly
% at the filtered dq current without a redundant abc-to-dq round trip.
Jrot = [0 -1; 1 0];
Bs = Bd*Rpark*Bs_TI;
deltaIdqBase = (Ad-eye(2))*idiqState+fd;
deltaIabcBase = Tdq2abc*(deltaIdqBase+Jrot*idiqState*(wel*Ts));
deltaIabcSwitch = Tdq2abc*Bs;

if predictionValid
    predictionError = iabcReconstruction-iabcPredictedPrevious;
else
    predictionError = zeros(3,1);
end
reconstructionError = Iabc_Motor-iabcReconstruction;
Tclarke = [2/3, -1/3, -1/3; ...
           0, 1/sqrt(3), -1/sqrt(3)];
predictionError_dq = Rpark*(Tclarke*predictionError);
reconstructionError_dq = Rpark*(Tclarke*reconstructionError);
iabcAverageEstimated = iabcReconstruction;
iabcRippleEstimated = zeros(3,1);
rippleResidual = zeros(3,1);
iabcSwitchCorrectionRaw = zeros(3,1);
end

== matlab function FCSMPC_double_vector_2025b/FCS_MPC/BuildModel/BuildModel/QP_Precompute_10k_Simplified ==
  data: Ld input double size=[1 1]; H output double size=[15 15]; Lq input double size=[1 1]; Rs input double size=[1 1]; Psi input double size=[1 1]; wel input double size=[1 1]; Ts input double size=[1 1]; Vdc input double size=[1 1]; lambda_fsw input double size=[1 1]; Sin_Cos_Theta input double size=[2 1]; filterTimeConstant input double size=[1 1]; sensorTimeConstant input double size=[1 1]; Gamma output double size=[10 2]; Phi output double size=[10 1]; Lambdafsw_SE output double size=[15 3]; Upsil output double size=[10 15]; Bd output double size=[2 2]; Bs_TI output double size=[2 3]; deltaIdqBaseOffset output double size=[2 1]; deltaIdqState output double size=[2 2]; magnitudeGain output double size=[1 1]; phaseCompensation output double size=[2 2]; rippleAttenuation output double size=[1 1]; rippleDelay output double size=[1 1]
function [H,Gamma,Phi,Lambdafsw_SE,Upsil, ...
    Bd,Bs_TI,deltaIdqBaseOffset,deltaIdqState, ...
    magnitudeGain,phaseCompensation,rippleAttenuation,rippleDelay] = ...
    QP_Precompute_10k_Simplified( ...
    Ld,Lq,Rs,Psi,wel,Ts,Vdc,lambda_fsw,Sin_Cos_Theta, ...
    filterTimeConstant,sensorTimeConstant)
%#codegen
% Slow-rate model/QP preparation. The midpoint angle theta+wel*50 us is
% used only to freeze the QP Hessian/Upsil over the 100-us interval.
% Instantaneous current transforms and switching-current increments are
% deliberately rebuilt from the current angle in QP_Runtime_40k_Simplified.

Np = 5;
nu = 3;
ny = 2;
Ts = max(realmin('double'),double(Ts));
filterTimeConstant = max(0.0,double(filterTimeConstant));
sensorTimeConstant = max(0.0,double(sensorTimeConstant));

Ac = [-Rs/Ld, wel*Lq/Ld; -wel*Ld/Lq, -Rs/Lq];
Bc = [1/Ld, 0; 0, 1/Lq];
fc = [0; -wel*Psi/Lq];
M = [Ac, Bc, fc; zeros(3,5)];
Md = expm(M*Ts);
Ad = Md(1:2,1:2);
Bd = Md(1:2,3:4);
fd = Md(1:2,5);

Apow = zeros(ny*(Np+1),ny);
Apow(1:ny,:) = eye(ny);
for m = 1:Np
    Apow(m*ny+(1:ny),:) = Apow((m-1)*ny+(1:ny),:)*Ad;
end

Gamma = zeros(ny*Np,ny);
Phi = zeros(ny*Np,1);
for i = 1:Np
    rows = (i-1)*ny+(1:ny);
    Gamma(rows,:) = Apow(i*ny+(1:ny),:);
    acc = zeros(ny,1);
    for m = 0:i-1
        acc = acc+Apow(m*ny+(1:ny),:)*fd;
    end
    Phi(rows) = acc;
end

S = eye(nu*Np);
for i = 2:Np
    S((i-1)*nu+(1:nu),(i-2)*nu+(1:nu)) = -eye(nu);
end
E = [eye(nu); zeros(nu*(Np-1),nu)];
lambdaEffective = max(lambda_fsw,1.0e-6);
Lambdafsw_SE = lambdaEffective*(S.'*E);
Lambdafsw_Ssquare = lambdaEffective*(S.'*S);

% One common midpoint electrical angle for the entire controller model.
sinTheta = Sin_Cos_Theta(1);
cosTheta = Sin_Cos_Theta(2);
deltaTheta = wel*50.0e-6;
sinDelta = sin(deltaTheta);
cosDelta = cos(deltaTheta);
sinMid = sinTheta*cosDelta+cosTheta*sinDelta;
cosMid = cosTheta*cosDelta-sinTheta*sinDelta;
RpMid = [cosMid, sinMid; -sinMid, cosMid];
Msw = eye(3)-ones(3)/3;
Tc = (2/3)*[1, -1/2, -1/2; 0, sqrt(3)/2, -sqrt(3)/2];
Bs_TI = Tc*Vdc*Msw;
deltaIdqSwitchMid = Bd*RpMid*Bs_TI;
Jrot = [0 -1; 1 0];
deltaIdqState = Ad-eye(2)+Jrot*(wel*Ts);
deltaIdqBaseOffset = fd;

Upsil = zeros(ny*Np,nu*Np);
for i = 1:Np
    rows = (i-1)*ny+(1:ny);
    for j = 1:i
        cols = (j-1)*nu+(1:nu);
        Upsil(rows,cols) = Apow((i-j)*ny+(1:ny),:)*deltaIdqSwitchMid;
    end
end

W = Upsil.'*Upsil+Lambdafsw_Ssquare;
W = 0.5*(W+W.');
W = W+1.0e-12*max(1.0,norm(W,'fro'))*eye(nu*Np);
Jx = fliplr(eye(nu*Np));
[Rt,p] = chol(Jx*W*Jx);
if p ~= 0
    error('H is not positive definite. Increase lambda_sw.');
end
H = Jx*Rt*Jx;

% Angle/frequency-related filter coefficients are also slow-rate values.
omegaFilter = wel*filterTimeConstant;
omegaSensor = wel*sensorTimeConstant;
magnitudeGain = sqrt(1.0+omegaFilter*omegaFilter)* ...
    sqrt(1.0+omegaSensor*omegaSensor);
w = abs(wel);
if w > 1.0e-6
    basePhaseDelay = (atan(w*filterTimeConstant)+ ...
        atan(w*sensorTimeConstant))/w;
else
    basePhaseDelay = filterTimeConstant+sensorTimeConstant;
end
phase = wel*basePhaseDelay;
phaseCompensation = [cos(phase), -sin(phase); sin(phase), cos(phase)];

omegaRipple = 2.0*pi*17.0e3;
xFilter = omegaRipple*filterTimeConstant;
xSensor = omegaRipple*sensorTimeConstant;
rippleAttenuation = 1.0/(sqrt(1.0+xFilter*xFilter)* ...
    sqrt(1.0+xSensor*xSensor));
rippleDelay = (atan(xFilter)+atan(xSensor))/omegaRipple;
rippleDelay = min(max(0.0,rippleDelay),2.0*Ts);
end
